simulink model "MotionControl"  (R2026b)
settings: Solver=VariableStepAuto
undefined symbols (not defined in the file): motionCfg, profileCfg
libraries: DiscretePID x1
settings Model: Creator=24322  LastModifiedBy=24322

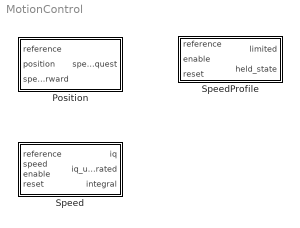
== system MotionControl ==
  Position : Subsystem
  Speed : Subsystem
  SpeedProfile : Subsystem  mask{profileCfg=profileCfg}
      mask prompts: profileCfg "Discrete speed profile configuration"

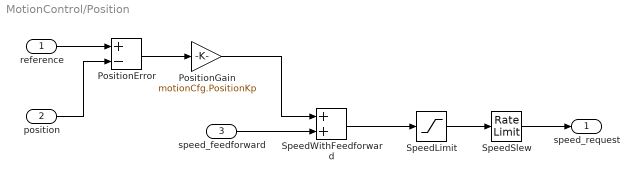
== system MotionControl/Position ==
  reference : Inport
  position : Inport  Port=2
  speed_feedforward : Inport  Port=3
  PositionError : Sum  Inputs=+-
  PositionGain : Gain  Gain=motionCfg.PositionKp
  SpeedLimit : Saturate  UpperLimit=motionCfg.SpeedLimit  LowerLimit=-motionCfg.SpeedLimit
  SpeedSlew : RateLimiter  RisingSlewLimit=motionCfg.AccelerationLimit  FallingSlewLimit=-motionCfg.AccelerationLimit  SampleTimeMode=inherited
  SpeedWithFeedforward : Sum
  speed_request : Outport
  wires:
  SpeedSlew/1 -> speed_request/1
  SpeedLimit/1 -> SpeedSlew/1
  SpeedWithFeedforward/1 -> SpeedLimit/1
  speed_feedforward/1 -> SpeedWithFeedforward/2
  PositionGain/1 -> SpeedWithFeedforward/1
  PositionError/1 -> PositionGain/1
  position/1 -> PositionError/2
  reference/1 -> PositionError/1

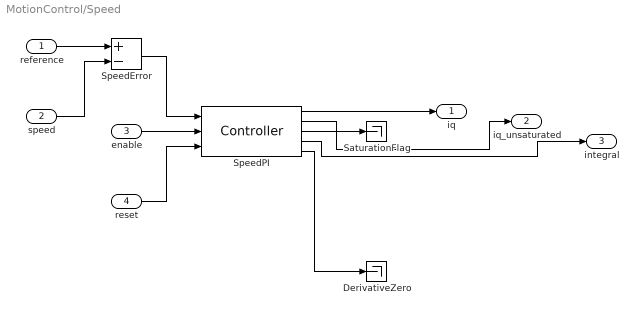
== system MotionControl/Speed ==
  reference : Inport
  speed : Inport  Port=2
  enable : Inport  Port=3
  reset : Inport  Port=4
  DerivativeZero : Terminator
  SaturationFlag : Terminator
  SpeedError : Sum  Inputs=+-
  SpeedPI : DiscretePID/Controller  Kp=motionCfg.Kp  Ki=motionCfg.Ki  Ts=motionCfg.Ts  UMin=-motionCfg.CurrentLimit  UMax=motionCfg.CurrentLimit  X0=0  Kaw=motionCfg.Kaw  Kd=0  Tf=motionCfg.Ts
  iq : Outport
  iq_unsaturated : Outport  Port=2
  integral : Outport  Port=3
  wires:
  SpeedPI/5 -> DerivativeZero/1
  SpeedPI/4 -> integral/1
  SpeedPI/3 -> SaturationFlag/1
  SpeedPI/2 -> iq_unsaturated/1
  SpeedPI/1 -> iq/1
  reset/1 -> SpeedPI/3
  enable/1 -> SpeedPI/2
  SpeedError/1 -> SpeedPI/1
  speed/1 -> SpeedError/2
  reference/1 -> SpeedError/1

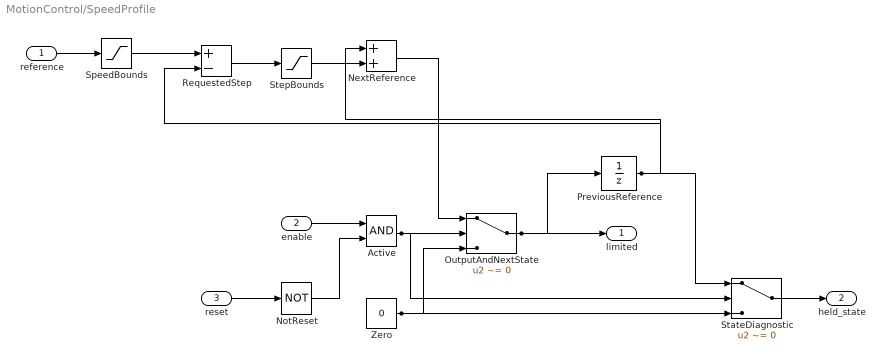
== system MotionControl/SpeedProfile ==
  reference : Inport  SampleTime=profileCfg.Ts
  enable : Inport  Port=2  SampleTime=profileCfg.Ts
  reset : Inport  Port=3  SampleTime=profileCfg.Ts
  Active : Logic  IconShape=distinctive  AllPortsSameDT=off  OutDataTypeStr=boolean
  NextReference : Sum
  NotReset : Logic  Operator=NOT  IconShape=distinctive  AllPortsSameDT=off  OutDataTypeStr=boolean
  OutputAndNextState : Switch  Criteria=u2 ~= 0  SaturateOnIntegerOverflow=off  InputSameDT=off
  PreviousReference : UnitDelay  SampleTime=profileCfg.Ts
  RequestedStep : Sum  Inputs=+-
  SpeedBounds : Saturate  UpperLimit=profileCfg.Maximum  LowerLimit=profileCfg.Minimum
  StateDiagnostic : Switch  Criteria=u2 ~= 0  SaturateOnIntegerOverflow=off  InputSameDT=off
  StepBounds : Saturate  UpperLimit=profileCfg.RisingStep  LowerLimit=-profileCfg.FallingStep
  Zero : Constant  Value=0
  limited : Outport
  held_state : Outport  Port=2
  wires:
  StateDiagnostic/1 -> held_state/1
  OutputAndNextState/1 -> PreviousReference/1, limited/1
  Zero/1 -> OutputAndNextState/3, StateDiagnostic/3
  Active/1 -> OutputAndNextState/2, StateDiagnostic/2
  NextReference/1 -> OutputAndNextState/1
  NotReset/1 -> Active/2
  enable/1 -> Active/1
  reset/1 -> NotReset/1
  StepBounds/1 -> NextReference/2
  RequestedStep/1 -> StepBounds/1
  PreviousReference/1 -> NextReference/1, RequestedStep/2, StateDiagnostic/1
  SpeedBounds/1 -> RequestedStep/1
  reference/1 -> SpeedBounds/1
